simulink model "talos_navigation"  (R2023a)
settings: Solver=FixedStepDiscrete  StartTime=0.0  StopTime=10.0  FixedStep=1/1000.0  RelTol=1e-3  EnableMultiTasking=on
undefined symbols (not defined in the file): accel, child_frame_id, child_frame_id_SL_Info, data, data_SL_Info, header, layout, transform, transforms, transforms_SL_Info
libraries: ros2lib x187, simulink x9, sharedTrackingLibrary x1
(part 2 of 3)

== system talos_navigation/Parameters/estimator ==
  estimator_bus : BusCreator  Inputs=17  OutDataTypeStr=Bus: talos_nav_params_estimator  NonVirtualBus=on
  gravitational_acceleration : ros2lib/Get Parameter  ParameterName=navigation__estimator__gravitational_acceleration  ParameterType=double  ParameterMaxArrayLength=16  ParameterInitialValue=9.8  SampleTime=1/10.0  ModelName=ros2lib  BlockId=ParamGet_ros2lib_196
  imu_acceleration_bias : Subsystem
  imu_acceleration_bias_density : ros2lib/Get Parameter  ParameterName=navigation__estimator__imu_acceleration_bias_density  ParameterType=double  ParameterMaxArrayLength=16  ParameterInitialValue=1e-07  SampleTime=1/10.0  ModelName=ros2lib  BlockId=ParamGet_ros2lib_196
  imu_acceleration_bias_rotation_variance : ros2lib/Get Parameter  ParameterName=navigation__estimator__imu_acceleration_bias_rotation_variance  ParameterType=double  ParameterMaxArrayLength=16  ParameterInitialValue=0.0016  SampleTime=1/10.0  ModelName=ros2lib  BlockId=ParamGet_ros2lib_196
  imu_acceleration_bias_variance : ros2lib/Get Parameter  ParameterName=navigation__estimator__imu_acceleration_bias_variance  ParameterType=double  ParameterMaxArrayLength=16  ParameterInitialValue=0.0004  SampleTime=1/10.0  ModelName=ros2lib  BlockId=ParamGet_ros2lib_196
  imu_acceleration_update : ros2lib/Get Parameter  ParameterName=navigation__estimator__imu_acceleration_update  ParameterType=int64  ParameterMaxArrayLength=16  ParameterInitialValue=2  SampleTime=1/10.0  ModelName=talos_navigation  BlockId=ParamGet_talos_navigation_167
  imu_angular_acceleration_noise_bandwidth : ros2lib/Get Parameter  ParameterName=navigation__estimator__imu_angular_acceleration_noise_bandwidth  ParameterType=double  ParameterMaxArrayLength=16  ParameterInitialValue=40  SampleTime=1/10.0  ModelName=ros2lib  BlockId=ParamGet_ros2lib_196
  imu_angular_acceleration_time_constant : ros2lib/Get Parameter  ParameterName=navigation__estimator__imu_angular_acceleration_time_constant  ParameterType=double  ParameterMaxArrayLength=16  ParameterInitialValue=0.005  SampleTime=1/10.0  ModelName=ros2lib  BlockId=ParamGet_ros2lib_196
  imu_quaternion_norm_tolerance : ros2lib/Get Parameter  ParameterName=navigation__estimator__imu_quaternion_norm_tolerance  ParameterType=double  ParameterMaxArrayLength=16  ParameterInitialValue=0.01  SampleTime=1/10.0  ModelName=ros2lib  BlockId=ParamGet_ros2lib_196
  imu_yaw_rate_fallback : ros2lib/Get Parameter  ParameterName=navigation__estimator__imu_yaw_rate_fallback  ParameterType=boolean  ParameterMaxArrayLength=16  ParameterInitialValue=1  SampleTime=1/10.0  ModelName=talos_navigation  BlockId=ParamGet_talos_navigation_219
  imu_yaw_rate_fallback_variance : ros2lib/Get Parameter  ParameterName=navigation__estimator__imu_yaw_rate_fallback_variance  ParameterType=double  ParameterMaxArrayLength=16  ParameterInitialValue=0.0001  SampleTime=1/10.0  ModelName=ros2lib  BlockId=ParamGet_ros2lib_196
  initial_quaternion_tolerance : ros2lib/Get Parameter  ParameterName=navigation__estimator__initial_quaternion_tolerance  ParameterType=double  ParameterMaxArrayLength=16  ParameterInitialValue=0.001  SampleTime=1/10.0  ModelName=ros2lib  BlockId=ParamGet_ros2lib_196
  initialize_tilt_from_imu : ros2lib/Get Parameter  ParameterName=navigation__estimator__initialize_tilt_from_imu  ParameterType=boolean  ParameterMaxArrayLength=16  ParameterInitialValue=1  SampleTime=1/10.0  ModelName=talos_navigation  BlockId=ParamGet_talos_navigation_165
  process_noise_diag : Subsystem
  reset_covariance_diag : Subsystem
  scalar_fog_correction : ros2lib/Get Parameter  ParameterName=navigation__estimator__scalar_fog_correction  ParameterType=boolean  ParameterMaxArrayLength=16  ParameterInitialValue=1  SampleTime=1/10.0  ModelName=talos_navigation  BlockId=ParamGet_talos_navigation_222
  vectornav_tilt_correction_frequency : ros2lib/Get Parameter  ParameterName=navigation__estimator__vectornav_tilt_correction_frequency  ParameterType=double  ParameterMaxArrayLength=16  ParameterInitialValue=0  SampleTime=1/10.0  ModelName=ros2lib  BlockId=ParamGet_ros2lib_196
  estimator : Outport
  wires:
  initialize_tilt_from_imu/1 -> estimator_bus/1  "initialize_tilt_from_imu"
  vectornav_tilt_correction_frequency/1 -> estimator_bus/2  "vectornav_tilt_correction_frequency"
  imu_acceleration_update/1 -> estimator_bus/3  "imu_acceleration_update"
  gravitational_acceleration/1 -> estimator_bus/4  "gravitational_acceleration"
  imu_acceleration_bias/1(value) -> estimator_bus/5  "imu_acceleration_bias"
  imu_acceleration_bias_density/1 -> estimator_bus/6  "imu_acceleration_bias_density"
  imu_acceleration_bias_variance/1 -> estimator_bus/7  "imu_acceleration_bias_variance"
  imu_acceleration_bias_rotation_variance/1 -> estimator_bus/8  "imu_acceleration_bias_rotation_variance"
  imu_angular_acceleration_time_constant/1 -> estimator_bus/9  "imu_angular_acceleration_time_constant"
  imu_angular_acceleration_noise_bandwidth/1 -> estimator_bus/10  "imu_angular_acceleration_noise_bandwidth"
  process_noise_diag/1(value) -> estimator_bus/11  "process_noise_diag"
  reset_covariance_diag/1(value) -> estimator_bus/12  "reset_covariance_diag"
  initial_quaternion_tolerance/1 -> estimator_bus/13  "initial_quaternion_tolerance"
  imu_yaw_rate_fallback/1 -> estimator_bus/14  "imu_yaw_rate_fallback"
  imu_yaw_rate_fallback_variance/1 -> estimator_bus/15  "imu_yaw_rate_fallback_variance"
  imu_quaternion_norm_tolerance/1 -> estimator_bus/16  "imu_quaternion_norm_tolerance"
  scalar_fog_correction/1 -> estimator_bus/17  "scalar_fog_correction"
  estimator_bus/1 -> estimator/1

== system talos_navigation/Parameters/frames ==
  base_link_frame : ros2lib/Get Parameter  ParameterName=navigation__frames__base_link_frame  ParameterType=uint8[]  ParameterMaxArrayLength=64  ParameterInitialValue=0.0  SampleTime=1/10.0  ModelName=talos_navigation  BlockId=ParamGet_talos_navigation_7
  base_link_frame_length : Terminator
  dvl_frame_fallback : ros2lib/Get Parameter  ParameterName=navigation__frames__dvl_frame_fallback  ParameterType=uint8[]  ParameterMaxArrayLength=64  ParameterInitialValue=0.0  SampleTime=1/10.0  ModelName=talos_navigation  BlockId=ParamGet_talos_navigation_14
  dvl_frame_fallback_length : Terminator
  fog_frame_fallback : ros2lib/Get Parameter  ParameterName=navigation__frames__fog_frame_fallback  ParameterType=uint8[]  ParameterMaxArrayLength=64  ParameterInitialValue=0.0  SampleTime=1/10.0  ModelName=talos_navigation  BlockId=ParamGet_talos_navigation_12
  fog_frame_fallback_length : Terminator
  frames_bus : BusCreator  Inputs=6  OutDataTypeStr=Bus: talos_nav_params_frames  NonVirtualBus=on
  imu_frame_fallback : ros2lib/Get Parameter  ParameterName=navigation__frames__imu_frame_fallback  ParameterType=uint8[]  ParameterMaxArrayLength=64  ParameterInitialValue=0.0  SampleTime=1/10.0  ModelName=talos_navigation  BlockId=ParamGet_talos_navigation_10
  imu_frame_fallback_length : Terminator
  publish_tf : ros2lib/Get Parameter  ParameterName=navigation__frames__publish_tf  ParameterType=boolean  ParameterMaxArrayLength=16  ParameterInitialValue=1  SampleTime=1/10.0  ModelName=talos_navigation  BlockId=ParamGet_talos_navigation_9
  world_frame : ros2lib/Get Parameter  ParameterName=navigation__frames__world_frame  ParameterType=uint8[]  ParameterMaxArrayLength=64  ParameterInitialValue=0.0  SampleTime=1/10.0  ModelName=talos_navigation  BlockId=ParamGet_talos_navigation_5
  world_frame_length : Terminator
  frames : Outport
  wires:
  world_frame/2 -> world_frame_length/1
  world_frame/1 -> frames_bus/1  "world_frame"
  base_link_frame/2 -> base_link_frame_length/1
  base_link_frame/1 -> frames_bus/2  "base_link_frame"
  publish_tf/1 -> frames_bus/3  "publish_tf"
  imu_frame_fallback/2 -> imu_frame_fallback_length/1
  imu_frame_fallback/1 -> frames_bus/4  "imu_frame_fallback"
  fog_frame_fallback/2 -> fog_frame_fallback_length/1
  fog_frame_fallback/1 -> frames_bus/5  "fog_frame_fallback"
  dvl_frame_fallback/2 -> dvl_frame_fallback_length/1
  dvl_frame_fallback/1 -> frames_bus/6  "dvl_frame_fallback"
  frames_bus/1 -> frames/1

== system talos_navigation/Parameters/gates ==
  depth_rejection_threshold : ros2lib/Get Parameter  ParameterName=navigation__gates__depth_rejection_threshold  ParameterType=double  ParameterMaxArrayLength=16  ParameterInitialValue=5  SampleTime=1/10.0  ModelName=ros2lib  BlockId=ParamGet_ros2lib_196
  dvl_frozen_sample_limit : ros2lib/Get Parameter  ParameterName=navigation__gates__dvl_frozen_sample_limit  ParameterType=int64  ParameterMaxArrayLength=16  ParameterInitialValue=4  SampleTime=1/10.0  ModelName=talos_navigation  BlockId=ParamGet_talos_navigation_240
  dvl_rejection_threshold : ros2lib/Get Parameter  ParameterName=navigation__gates__dvl_rejection_threshold  ParameterType=double  ParameterMaxArrayLength=16  ParameterInitialValue=5  SampleTime=1/10.0  ModelName=ros2lib  BlockId=ParamGet_ros2lib_196
  dvl_sigma_jump_ratio : ros2lib/Get Parameter  ParameterName=navigation__gates__dvl_sigma_jump_ratio  ParameterType=double  ParameterMaxArrayLength=16  ParameterInitialValue=2  SampleTime=1/10.0  ModelName=ros2lib  BlockId=ParamGet_ros2lib_196
  dvl_sigma_min_history : ros2lib/Get Parameter  ParameterName=navigation__gates__dvl_sigma_min_history  ParameterType=int64  ParameterMaxArrayLength=16  ParameterInitialValue=8  SampleTime=1/10.0  ModelName=talos_navigation  BlockId=ParamGet_talos_navigation_242
  fog_rejection_threshold : ros2lib/Get Parameter  ParameterName=navigation__gates__fog_rejection_threshold  ParameterType=double  ParameterMaxArrayLength=16  ParameterInitialValue=0  SampleTime=1/10.0  ModelName=ros2lib  BlockId=ParamGet_ros2lib_196
  fog_vn_rate_tolerance : ros2lib/Get Parameter  ParameterName=navigation__gates__fog_vn_rate_tolerance  ParameterType=double  ParameterMaxArrayLength=16  ParameterInitialValue=0.05  SampleTime=1/10.0  ModelName=ros2lib  BlockId=ParamGet_ros2lib_196
  gate_consistency_stddev : Subsystem
  gate_consistency_threshold : ros2lib/Get Parameter  ParameterName=navigation__gates__gate_consistency_threshold  ParameterType=double  ParameterMaxArrayLength=16  ParameterInitialValue=2.5  SampleTime=1/10.0  ModelName=ros2lib  BlockId=ParamGet_ros2lib_196
  gate_flap_factor : ros2lib/Get Parameter  ParameterName=navigation__gates__gate_flap_factor  ParameterType=double  ParameterMaxArrayLength=16  ParameterInitialValue=4  SampleTime=1/10.0  ModelName=ros2lib  BlockId=ParamGet_ros2lib_196
  gate_min_recovery_window : ros2lib/Get Parameter  ParameterName=navigation__gates__gate_min_recovery_window  ParameterType=double  ParameterMaxArrayLength=16  ParameterInitialValue=0.25  SampleTime=1/10.0  ModelName=ros2lib  BlockId=ParamGet_ros2lib_196
  gate_reacquire_max_scale : ros2lib/Get Parameter  ParameterName=navigation__gates__gate_reacquire_max_scale  ParameterType=double  ParameterMaxArrayLength=16  ParameterInitialValue=4  SampleTime=1/10.0  ModelName=ros2lib  BlockId=ParamGet_ros2lib_196
  gate_reacquire_samples : ros2lib/Get Parameter  ParameterName=navigation__gates__gate_reacquire_samples  ParameterType=int64  ParameterMaxArrayLength=16  ParameterInitialValue=4  SampleTime=1/10.0  ModelName=talos_navigation  BlockId=ParamGet_talos_navigation_245
  gate_recovery_samples : ros2lib/Get Parameter  ParameterName=navigation__gates__gate_recovery_samples  ParameterType=int64  ParameterMaxArrayLength=16  ParameterInitialValue=5  SampleTime=1/10.0  ModelName=talos_navigation  BlockId=ParamGet_talos_navigation_246
  gate_recovery_time : ros2lib/Get Parameter  ParameterName=navigation__gates__gate_recovery_time  ParameterType=double  ParameterMaxArrayLength=16  ParameterInitialValue=0.5  SampleTime=1/10.0  ModelName=ros2lib  BlockId=ParamGet_ros2lib_196
  gates_bus : BusCreator  Inputs=17  OutDataTypeStr=Bus: talos_nav_params_gates  NonVirtualBus=on
  tilt_rejection_threshold : ros2lib/Get Parameter  ParameterName=navigation__gates__tilt_rejection_threshold  ParameterType=double  ParameterMaxArrayLength=16  ParameterInitialValue=10  SampleTime=1/10.0  ModelName=ros2lib  BlockId=ParamGet_ros2lib_196
  vn_rate_pairing_window : ros2lib/Get Parameter  ParameterName=navigation__gates__vn_rate_pairing_window  ParameterType=double  ParameterMaxArrayLength=16  ParameterInitialValue=0.01  SampleTime=1/10.0  ModelName=ros2lib  BlockId=ParamGet_ros2lib_196
  gates : Outport
  wires:
  dvl_rejection_threshold/1 -> gates_bus/1  "dvl_rejection_threshold"
  depth_rejection_threshold/1 -> gates_bus/2  "depth_rejection_threshold"
  tilt_rejection_threshold/1 -> gates_bus/3  "tilt_rejection_threshold"
  fog_rejection_threshold/1 -> gates_bus/4  "fog_rejection_threshold"
  fog_vn_rate_tolerance/1 -> gates_bus/5  "fog_vn_rate_tolerance"
  vn_rate_pairing_window/1 -> gates_bus/6  "vn_rate_pairing_window"
  gate_recovery_time/1 -> gates_bus/7  "gate_recovery_time"
  gate_consistency_stddev/1(value) -> gates_bus/8  "gate_consistency_stddev"
  dvl_frozen_sample_limit/1 -> gates_bus/9  "dvl_frozen_sample_limit"
  dvl_sigma_jump_ratio/1 -> gates_bus/10  "dvl_sigma_jump_ratio"
  dvl_sigma_min_history/1 -> gates_bus/11  "dvl_sigma_min_history"
  gate_reacquire_max_scale/1 -> gates_bus/12  "gate_reacquire_max_scale"
  gate_consistency_threshold/1 -> gates_bus/13  "gate_consistency_threshold"
  gate_reacquire_samples/1 -> gates_bus/14  "gate_reacquire_samples"
  gate_recovery_samples/1 -> gates_bus/15  "gate_recovery_samples"
  gate_min_recovery_window/1 -> gates_bus/16  "gate_min_recovery_window"
  gate_flap_factor/1 -> gates_bus/17  "gate_flap_factor"
  gates_bus/1 -> gates/1

== system talos_navigation/Parameters/mounts ==
  depth_frame : ros2lib/Get Parameter  ParameterName=navigation__mounts__depth_frame  ParameterType=uint8[]  ParameterMaxArrayLength=64  ParameterInitialValue=0.0  SampleTime=1/10.0  ModelName=talos_navigation  BlockId=ParamGet_talos_navigation_62
  depth_frame_length : Terminator
  depth_mount_valid : ros2lib/Get Parameter  ParameterName=navigation__mounts__depth_mount_valid  ParameterType=boolean  ParameterMaxArrayLength=16  ParameterInitialValue=0  SampleTime=1/10.0  ModelName=talos_navigation  BlockId=ParamGet_talos_navigation_64
  depth_rotation : Subsystem
  depth_translation : Subsystem
  dvl_mount_valid : ros2lib/Get Parameter  ParameterName=navigation__mounts__dvl_mount_valid  ParameterType=boolean  ParameterMaxArrayLength=16  ParameterInitialValue=0  SampleTime=1/10.0  ModelName=talos_navigation  BlockId=ParamGet_talos_navigation_48
  dvl_rotation : Subsystem
  dvl_translation : Subsystem
  fog_mount_valid : ros2lib/Get Parameter  ParameterName=navigation__mounts__fog_mount_valid  ParameterType=boolean  ParameterMaxArrayLength=16  ParameterInitialValue=0  SampleTime=1/10.0  ModelName=talos_navigation  BlockId=ParamGet_talos_navigation_34
  fog_rotation : Subsystem
  fog_translation : Subsystem
  imu_mount_valid : ros2lib/Get Parameter  ParameterName=navigation__mounts__imu_mount_valid  ParameterType=boolean  ParameterMaxArrayLength=16  ParameterInitialValue=0  SampleTime=1/10.0  ModelName=talos_navigation  BlockId=ParamGet_talos_navigation_20
  imu_rotation : Subsystem
  imu_translation : Subsystem
  mounts_bus : BusCreator  Inputs=14  OutDataTypeStr=Bus: talos_nav_params_mounts  NonVirtualBus=on
  parameters_loaded : ros2lib/Get Parameter  ParameterName=navigation__mounts__parameters_loaded  ParameterType=boolean  ParameterMaxArrayLength=16  ParameterInitialValue=0  SampleTime=1/10.0  ModelName=talos_navigation  BlockId=ParamGet_talos_navigation_19
  mounts : Outport
  wires:
  parameters_loaded/1 -> mounts_bus/1  "parameters_loaded"
  imu_mount_valid/1 -> mounts_bus/2  "imu_mount_valid"
  imu_translation/1(value) -> mounts_bus/3  "imu_translation"
  imu_rotation/1(value) -> mounts_bus/4  "imu_rotation"
  fog_mount_valid/1 -> mounts_bus/5  "fog_mount_valid"
  fog_translation/1(value) -> mounts_bus/6  "fog_translation"
  fog_rotation/1(value) -> mounts_bus/7  "fog_rotation"
  dvl_mount_valid/1 -> mounts_bus/8  "dvl_mount_valid"
  dvl_translation/1(value) -> mounts_bus/9  "dvl_translation"
  dvl_rotation/1(value) -> mounts_bus/10  "dvl_rotation"
  depth_frame/2 -> depth_frame_length/1
  depth_frame/1 -> mounts_bus/11  "depth_frame"
  depth_mount_valid/1 -> mounts_bus/12  "depth_mount_valid"
  depth_translation/1(value) -> mounts_bus/13  "depth_translation"
  depth_rotation/1(value) -> mounts_bus/14  "depth_rotation"
  mounts_bus/1 -> mounts/1

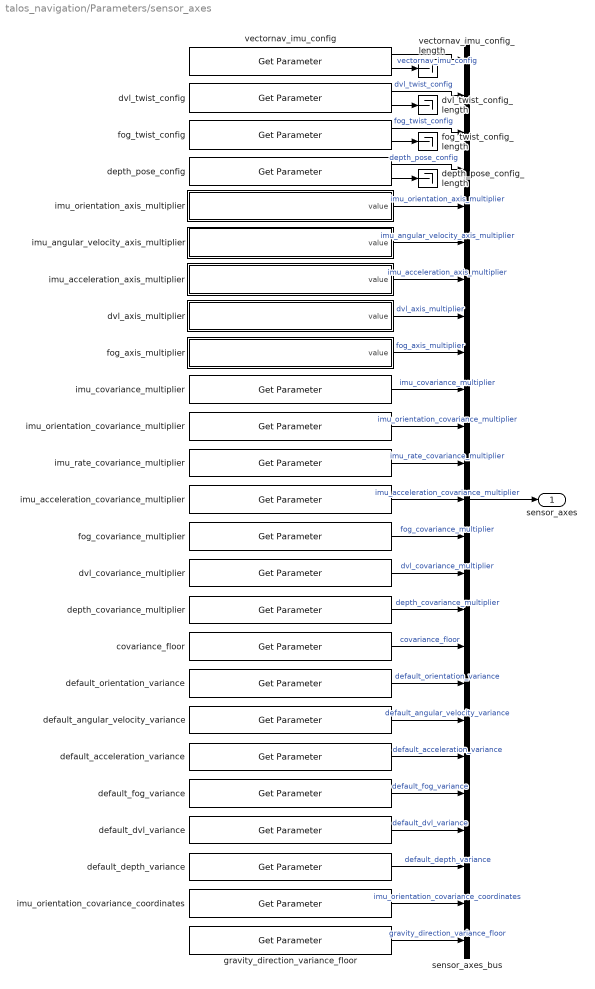
== system talos_navigation/Parameters/sensor_axes ==
  covariance_floor : ros2lib/Get Parameter  ParameterName=navigation__sensor_axes__covariance_floor  ParameterType=double  ParameterMaxArrayLength=16  ParameterInitialValue=1e-09  SampleTime=1/10.0  ModelName=ros2lib  BlockId=ParamGet_ros2lib_196
  default_acceleration_variance : ros2lib/Get Parameter  ParameterName=navigation__sensor_axes__default_acceleration_variance  ParameterType=double  ParameterMaxArrayLength=16  ParameterInitialValue=0.002  SampleTime=1/10.0  ModelName=ros2lib  BlockId=ParamGet_ros2lib_196
  default_angular_velocity_variance : ros2lib/Get Parameter  ParameterName=navigation__sensor_axes__default_angular_velocity_variance  ParameterType=double  ParameterMaxArrayLength=16  ParameterInitialValue=2e-05  SampleTime=1/10.0  ModelName=ros2lib  BlockId=ParamGet_ros2lib_196
  default_depth_variance : ros2lib/Get Parameter  ParameterName=navigation__sensor_axes__default_depth_variance  ParameterType=double  ParameterMaxArrayLength=16  ParameterInitialValue=0.0025  SampleTime=1/10.0  ModelName=ros2lib  BlockId=ParamGet_ros2lib_196
  default_dvl_variance : ros2lib/Get Parameter  ParameterName=navigation__sensor_axes__default_dvl_variance  ParameterType=double  ParameterMaxArrayLength=16  ParameterInitialValue=0.00025  SampleTime=1/10.0  ModelName=ros2lib  BlockId=ParamGet_ros2lib_196
  default_fog_variance : ros2lib/Get Parameter  ParameterName=navigation__sensor_axes__default_fog_variance  ParameterType=double  ParameterMaxArrayLength=16  ParameterInitialValue=1e-06  SampleTime=1/10.0  ModelName=ros2lib  BlockId=ParamGet_ros2lib_196
  default_orientation_variance : ros2lib/Get Parameter  ParameterName=navigation__sensor_axes__default_orientation_variance  ParameterType=double  ParameterMaxArrayLength=16  ParameterInitialValue=0.0002  SampleTime=1/10.0  ModelName=ros2lib  BlockId=ParamGet_ros2lib_196
  depth_covariance_multiplier : ros2lib/Get Parameter  ParameterName=navigation__sensor_axes__depth_covariance_multiplier  ParameterType=double  ParameterMaxArrayLength=16  ParameterInitialValue=1  SampleTime=1/10.0  ModelName=ros2lib  BlockId=ParamGet_ros2lib_196
  depth_pose_config : ros2lib/Get Parameter  ParameterName=navigation__sensor_axes__depth_pose_config  ParameterType=boolean[]  ParameterMaxArrayLength=15  ParameterInitialValue=[0;0;1;0;0;0;0;0;0;0;0;0;0;0;0]  SampleTime=1/10.0  ModelName=talos_navigation  BlockId=ParamGet_talos_navigation_114
  depth_pose_config_length : Terminator
  dvl_axis_multiplier : Subsystem
  dvl_covariance_multiplier : ros2lib/Get Parameter  ParameterName=navigation__sensor_axes__dvl_covariance_multiplier  ParameterType=double  ParameterMaxArrayLength=16  ParameterInitialValue=1  SampleTime=1/10.0  ModelName=ros2lib  BlockId=ParamGet_ros2lib_196
  dvl_twist_config : ros2lib/Get Parameter  ParameterName=navigation__sensor_axes__dvl_twist_config  ParameterType=boolean[]  ParameterMaxArrayLength=15  ParameterInitialValue=[0;0;0;0;0;0;1;1;1;0;0;0;0;0;0]  SampleTime=1/10.0  ModelName=talos_navigation  BlockId=ParamGet_talos_navigation_110
  dvl_twist_config_length : Terminator
  fog_axis_multiplier : Subsystem
  fog_covariance_multiplier : ros2lib/Get Parameter  ParameterName=navigation__sensor_axes__fog_covariance_multiplier  ParameterType=double  ParameterMaxArrayLength=16  ParameterInitialValue=1  SampleTime=1/10.0  ModelName=ros2lib  BlockId=ParamGet_ros2lib_196
  fog_twist_config : ros2lib/Get Parameter  ParameterName=navigation__sensor_axes__fog_twist_config  ParameterType=boolean[]  ParameterMaxArrayLength=15  ParameterInitialValue=[0;0;0;0;0;0;0;0;0;0;0;1;0;0;0]  SampleTime=1/10.0  ModelName=talos_navigation  BlockId=ParamGet_talos_navigation_112
  fog_twist_config_length : Terminator
  gravity_direction_variance_floor : ros2lib/Get Parameter  ParameterName=navigation__sensor_axes__gravity_direction_variance_floor  ParameterType=double  ParameterMaxArrayLength=16  ParameterInitialValue=1e-09  SampleTime=1/10.0  ModelName=ros2lib  BlockId=ParamGet_ros2lib_196
  imu_acceleration_axis_multiplier : Subsystem
  imu_acceleration_covariance_multiplier : ros2lib/Get Parameter  ParameterName=navigation__sensor_axes__imu_acceleration_covariance_multiplier  ParameterType=double  ParameterMaxArrayLength=16  ParameterInitialValue=1  SampleTime=1/10.0  ModelName=ros2lib  BlockId=ParamGet_ros2lib_196
  imu_angular_velocity_axis_multiplier : Subsystem
  imu_covariance_multiplier : ros2lib/Get Parameter  ParameterName=navigation__sensor_axes__imu_covariance_multiplier  ParameterType=double  ParameterMaxArrayLength=16  ParameterInitialValue=1  SampleTime=1/10.0  ModelName=ros2lib  BlockId=ParamGet_ros2lib_196
  imu_orientation_axis_multiplier : Subsystem
  imu_orientation_covariance_coordinates : ros2lib/Get Parameter  ParameterName=navigation__sensor_axes__imu_orientation_covariance_coordinates  ParameterType=int64  ParameterMaxArrayLength=16  ParameterInitialValue=1  SampleTime=1/10.0  ModelName=talos_navigation  BlockId=ParamGet_talos_navigation_160
  imu_orientation_covariance_multiplier : ros2lib/Get Parameter  ParameterName=navigation__sensor_axes__imu_orientation_covariance_multiplier  ParameterType=double  ParameterMaxArrayLength=16  ParameterInitialValue=1  SampleTime=1/10.0  ModelName=ros2lib  BlockId=ParamGet_ros2lib_196
  imu_rate_covariance_multiplier : ros2lib/Get Parameter  ParameterName=navigation__sensor_axes__imu_rate_covariance_multiplier  ParameterType=double  ParameterMaxArrayLength=16  ParameterInitialValue=0.01  SampleTime=1/10.0  ModelName=ros2lib  BlockId=ParamGet_ros2lib_196
  sensor_axes_bus : BusCreator  Inputs=25  OutDataTypeStr=Bus: talos_nav_params_sensor_axes  NonVirtualBus=on
  vectornav_imu_config : ros2lib/Get Parameter  ParameterName=navigation__sensor_axes__vectornav_imu_config  ParameterType=boolean[]  ParameterMaxArrayLength=15  ParameterInitialValue=[0;0;0;1;1;0;0;0;0;1;1;0;1;1;1]  SampleTime=1/10.0  ModelName=talos_navigation  BlockId=ParamGet_talos_navigation_108
  vectornav_imu_config_length : Terminator
  sensor_axes : Outport
  wires:
  vectornav_imu_config/2 -> vectornav_imu_config_length/1
  vectornav_imu_config/1 -> sensor_axes_bus/1  "vectornav_imu_config"
  dvl_twist_config/2 -> dvl_twist_config_length/1
  dvl_twist_config/1 -> sensor_axes_bus/2  "dvl_twist_config"
  fog_twist_config/2 -> fog_twist_config_length/1
  fog_twist_config/1 -> sensor_axes_bus/3  "fog_twist_config"
  depth_pose_config/2 -> depth_pose_config_length/1
  depth_pose_config/1 -> sensor_axes_bus/4  "depth_pose_config"
  imu_orientation_axis_multiplier/1(value) -> sensor_axes_bus/5  "imu_orientation_axis_multiplier"
  imu_angular_velocity_axis_multiplier/1(value) -> sensor_axes_bus/6  "imu_angular_velocity_axis_multiplier"
  imu_acceleration_axis_multiplier/1(value) -> sensor_axes_bus/7  "imu_acceleration_axis_multiplier"
  dvl_axis_multiplier/1(value) -> sensor_axes_bus/8  "dvl_axis_multiplier"
  fog_axis_multiplier/1(value) -> sensor_axes_bus/9  "fog_axis_multiplier"
  imu_covariance_multiplier/1 -> sensor_axes_bus/10  "imu_covariance_multiplier"
  imu_orientation_covariance_multiplier/1 -> sensor_axes_bus/11  "imu_orientation_covariance_multiplier"
  imu_rate_covariance_multiplier/1 -> sensor_axes_bus/12  "imu_rate_covariance_multiplier"
  imu_acceleration_covariance_multiplier/1 -> sensor_axes_bus/13  "imu_acceleration_covariance_multiplier"
  fog_covariance_multiplier/1 -> sensor_axes_bus/14  "fog_covariance_multiplier"
  dvl_covariance_multiplier/1 -> sensor_axes_bus/15  "dvl_covariance_multiplier"
  depth_covariance_multiplier/1 -> sensor_axes_bus/16  "depth_covariance_multiplier"
  covariance_floor/1 -> sensor_axes_bus/17  "covariance_floor"
  default_orientation_variance/1 -> sensor_axes_bus/18  "default_orientation_variance"
  default_angular_velocity_variance/1 -> sensor_axes_bus/19  "default_angular_velocity_variance"
  default_acceleration_variance/1 -> sensor_axes_bus/20  "default_acceleration_variance"
  default_fog_variance/1 -> sensor_axes_bus/21  "default_fog_variance"
  default_dvl_variance/1 -> sensor_axes_bus/22  "default_dvl_variance"
  default_depth_variance/1 -> sensor_axes_bus/23  "default_depth_variance"
  imu_orientation_covariance_coordinates/1 -> sensor_axes_bus/24  "imu_orientation_covariance_coordinates"
  gravity_direction_variance_floor/1 -> sensor_axes_bus/25  "gravity_direction_variance_floor"
  sensor_axes_bus/1 -> sensor_axes/1

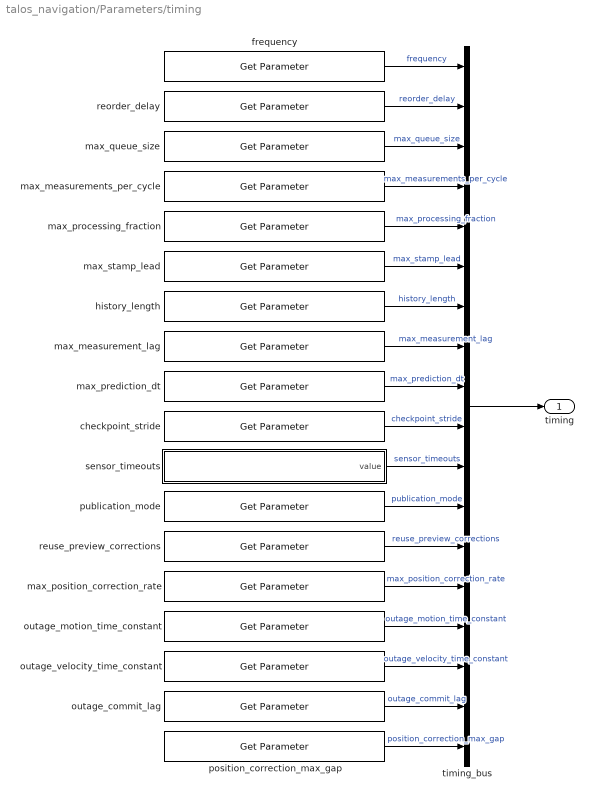
== system talos_navigation/Parameters/timing ==
  checkpoint_stride : ros2lib/Get Parameter  ParameterName=navigation__timing__checkpoint_stride  ParameterType=double  ParameterMaxArrayLength=16  ParameterInitialValue=0.005  SampleTime=1/10.0  ModelName=ros2lib  BlockId=ParamGet_ros2lib_196
  frequency : ros2lib/Get Parameter  ParameterName=navigation__timing__frequency  ParameterType=double  ParameterMaxArrayLength=16  ParameterInitialValue=30  SampleTime=1/10.0  ModelName=ros2lib  BlockId=ParamGet_ros2lib_196
  history_length : ros2lib/Get Parameter  ParameterName=navigation__timing__history_length  ParameterType=double  ParameterMaxArrayLength=16  ParameterInitialValue=0.5  SampleTime=1/10.0  ModelName=ros2lib  BlockId=ParamGet_ros2lib_196
  max_measurement_lag : ros2lib/Get Parameter  ParameterName=navigation__timing__max_measurement_lag  ParameterType=double  ParameterMaxArrayLength=16  ParameterInitialValue=2  SampleTime=1/10.0  ModelName=ros2lib  BlockId=ParamGet_ros2lib_196
  max_measurements_per_cycle : ros2lib/Get Parameter  ParameterName=navigation__timing__max_measurements_per_cycle  ParameterType=int64  ParameterMaxArrayLength=16  ParameterInitialValue=0  SampleTime=1/10.0  ModelName=talos_navigation  BlockId=ParamGet_talos_navigation_84
  max_position_correction_rate : ros2lib/Get Parameter  ParameterName=navigation__timing__max_position_correction_rate  ParameterType=double  ParameterMaxArrayLength=16  ParameterInitialValue=0.2  SampleTime=1/10.0  ModelName=ros2lib  BlockId=ParamGet_ros2lib_196
  max_prediction_dt : ros2lib/Get Parameter  ParameterName=navigation__timing__max_prediction_dt  ParameterType=double  ParameterMaxArrayLength=16  ParameterInitialValue=0.1  SampleTime=1/10.0  ModelName=ros2lib  BlockId=ParamGet_ros2lib_196
  max_processing_fraction : ros2lib/Get Parameter  ParameterName=navigation__timing__max_processing_fraction  ParameterType=double  ParameterMaxArrayLength=16  ParameterInitialValue=0.5  SampleTime=1/10.0  ModelName=ros2lib  BlockId=ParamGet_ros2lib_196
  max_queue_size : ros2lib/Get Parameter  ParameterName=navigation__timing__max_queue_size  ParameterType=int64  ParameterMaxArrayLength=16  ParameterInitialValue=512  SampleTime=1/10.0  ModelName=talos_navigation  BlockId=ParamGet_talos_navigation_83
  max_stamp_lead : ros2lib/Get Parameter  ParameterName=navigation__timing__max_stamp_lead  ParameterType=double  ParameterMaxArrayLength=16  ParameterInitialValue=1  SampleTime=1/10.0  ModelName=ros2lib  BlockId=ParamGet_ros2lib_196
  outage_commit_lag : ros2lib/Get Parameter  ParameterName=navigation__timing__outage_commit_lag  ParameterType=double  ParameterMaxArrayLength=16  ParameterInitialValue=1  SampleTime=1/10.0  ModelName=ros2lib  BlockId=ParamGet_ros2lib_196
  outage_motion_time_constant : ros2lib/Get Parameter  ParameterName=navigation__timing__outage_motion_time_constant  ParameterType=double  ParameterMaxArrayLength=16  ParameterInitialValue=0.5  SampleTime=1/10.0  ModelName=ros2lib  BlockId=ParamGet_ros2lib_196
  outage_velocity_time_constant : ros2lib/Get Parameter  ParameterName=navigation__timing__outage_velocity_time_constant  ParameterType=double  ParameterMaxArrayLength=16  ParameterInitialValue=2  SampleTime=1/10.0  ModelName=ros2lib  BlockId=ParamGet_ros2lib_196
  position_correction_max_gap : ros2lib/Get Parameter  ParameterName=navigation__timing__position_correction_max_gap  ParameterType=double  ParameterMaxArrayLength=16  ParameterInitialValue=1  SampleTime=1/10.0  ModelName=ros2lib  BlockId=ParamGet_ros2lib_196
  publication_mode : ros2lib/Get Parameter  ParameterName=navigation__timing__publication_mode  ParameterType=int64  ParameterMaxArrayLength=16  ParameterInitialValue=2  SampleTime=1/10.0  ModelName=talos_navigation  BlockId=ParamGet_talos_navigation_98
  reorder_delay : ros2lib/Get Parameter  ParameterName=navigation__timing__reorder_delay  ParameterType=double  ParameterMaxArrayLength=16  ParameterInitialValue=0.02  SampleTime=1/10.0  ModelName=ros2lib  BlockId=ParamGet_ros2lib_196
  reuse_preview_corrections : ros2lib/Get Parameter  ParameterName=navigation__timing__reuse_preview_corrections  ParameterType=boolean  ParameterMaxArrayLength=16  ParameterInitialValue=1  SampleTime=1/10.0  ModelName=talos_navigation  BlockId=ParamGet_talos_navigation_99
  sensor_timeouts : Subsystem
  timing_bus : BusCreator  Inputs=18  OutDataTypeStr=Bus: talos_nav_params_timing  NonVirtualBus=on
  timing : Outport
  wires:
  frequency/1 -> timing_bus/1  "frequency"
  reorder_delay/1 -> timing_bus/2  "reorder_delay"
  max_queue_size/1 -> timing_bus/3  "max_queue_size"
  max_measurements_per_cycle/1 -> timing_bus/4  "max_measurements_per_cycle"
  max_processing_fraction/1 -> timing_bus/5  "max_processing_fraction"
  max_stamp_lead/1 -> timing_bus/6  "max_stamp_lead"
  history_length/1 -> timing_bus/7  "history_length"
  max_measurement_lag/1 -> timing_bus/8  "max_measurement_lag"
  max_prediction_dt/1 -> timing_bus/9  "max_prediction_dt"
  checkpoint_stride/1 -> timing_bus/10  "checkpoint_stride"
  sensor_timeouts/1(value) -> timing_bus/11  "sensor_timeouts"
  publication_mode/1 -> timing_bus/12  "publication_mode"
  reuse_preview_corrections/1 -> timing_bus/13  "reuse_preview_corrections"
  max_position_correction_rate/1 -> timing_bus/14  "max_position_correction_rate"
  outage_motion_time_constant/1 -> timing_bus/15  "outage_motion_time_constant"
  outage_velocity_time_constant/1 -> timing_bus/16  "outage_velocity_time_constant"
  outage_commit_lag/1 -> timing_bus/17  "outage_commit_lag"
  position_correction_max_gap/1 -> timing_bus/18  "position_correction_max_gap"
  timing_bus/1 -> timing/1

== system talos_navigation/Publish_System/Acceleration ==
  enable : Inport
  time : Inport  Port=2
  base_id : Inport  Port=3
  base_length : Inport  Port=4
  x : Inport  Port=5
  accel_cov : Inport  Port=6
  blank : ros2lib/Blank Message  messageClass=Message  entityType=geometry_msgs/AccelWithCovarianceStamped  messageType=geometry_msgs/AccelWithCovarianceStamped  SampleTime=1/500.0
  fill : BusAssignment  AssignedSignals=header.stamp,header.frame_id,header.frame_id_SL_Info.CurrentLength,accel.accel.linear.x,accel.accel.linear.y,accel.accel.linear.z,accel.covariance
  fill_publish : Subsystem  TreatAsAtomicUnit=on
  x_elements : Demux  Outputs=3
  x_fields : Selector  InputPortWidth=19  IndexOptions=Index vector (dialog)  Indices=14:16  OutputSizes=1
  wires:
  blank/1 -> fill/1
  time/1 -> fill/2  "header.stamp"
  base_id/1 -> fill/3  "header.frame_id"
  base_length/1 -> fill/4  "frame_id_SL_Info.CurrentLength"
  x/1 -> x_fields/1
  x_fields/1 -> x_elements/1
  x_elements/1 -> fill/5  "linear.x"
  x_elements/2 -> fill/6  "linear.y"
  x_elements/3 -> fill/7  "linear.z"
  accel_cov/1 -> fill/8  "accel.covariance"
  fill/1 -> fill_publish/1(msg)  "msg"
  enable/1 -> fill_publish/Enable

== system talos_navigation/Publish_System/Base_Frame_ID ==
  name : Inport
  chars : Sum  Inputs=+  OutDataTypeStr=uint32
  count : DataTypeConversion  OutDataTypeStr=uint32  SaturateOnIntegerOverflow=off  RndMeth=Floor
  is_char : simulink/Logic and Bit Operations/Compare To Zero  relop=~=  OutDataTypeStr=boolean
  padded : Concatenate
  padding : Constant  Value=zeros(64, 1, 'uint8')
  frame_id : Outport
  length : Outport  Port=2
  wires:
  name/1 -> padded/1, is_char/1
  padding/1 -> padded/2
  padded/1 -> frame_id/1  "frame_id"
  is_char/1 -> count/1
  count/1 -> chars/1
  chars/1 -> length/1  "length"

== system talos_navigation/Publish_System/Diagnostics ==
  enable : Inport
  diag : Inport  Port=2
  part_0_blank : ros2lib/Blank Message  messageClass=Message  entityType=std_msgs/Float64MultiArray  messageType=std_msgs/Float64MultiArray  SampleTime=1/500.0
  part_0_fill : BusAssignment  AssignedSignals=data,data_SL_Info.CurrentLength,layout.data_offset
  part_0_length : Constant  Value=uint32(128)  OutDataTypeStr=uint32
  part_0_offset : Constant  Value=uint32(0)  OutDataTypeStr=uint32
  part_0_publish : Subsystem  TreatAsAtomicUnit=on
  part_0_values : Selector  InputPortWidth=162  IndexOptions=Starting index (dialog)  Indices=1  OutputSizes=128
  part_1_blank : ros2lib/Blank Message  messageClass=Message  entityType=std_msgs/Float64MultiArray  messageType=std_msgs/Float64MultiArray  SampleTime=1/500.0
  part_1_data : Concatenate
  part_1_fill : BusAssignment  AssignedSignals=data,data_SL_Info.CurrentLength,layout.data_offset
  part_1_length : Constant  Value=uint32(62)  OutDataTypeStr=uint32
  part_1_offset : Constant  Value=uint32(100)  OutDataTypeStr=uint32
  part_1_padding : Constant  Value=zeros(66, 1)
  part_1_publish : Subsystem  TreatAsAtomicUnit=on
  part_1_values : Selector  InputPortWidth=162  IndexOptions=Starting index (dialog)  Indices=101  OutputSizes=62
  wires:
  part_0_blank/1 -> part_0_fill/1
  part_0_length/1 -> part_0_fill/3  "length"
  part_0_offset/1 -> part_0_fill/4  "offset"
  [Diag] -> part_0_values/1
  part_0_values/1 -> part_0_fill/2  "data"
  part_0_fill/1 -> part_0_publish/1(msg)  "msg"
  enable/1 -> part_0_publish/Enable, part_1_publish/Enable
  part_1_blank/1 -> part_1_fill/1
  part_1_length/1 -> part_1_fill/3  "length"
  part_1_offset/1 -> part_1_fill/4  "offset"
  [Diag] -> part_1_values/1
  part_1_values/1 -> part_1_data/1
  part_1_padding/1 -> part_1_data/2
  part_1_data/1 -> part_1_fill/2  "data"
  part_1_fill/1 -> part_1_publish/1(msg)  "msg"
  diag/1 -> [Diag]

== system talos_navigation/Publish_System/Odometry ==
  enable : Inport
  time : Inport  Port=2
  world_id : Inport  Port=3
  world_length : Inport  Port=4
  base_id : Inport  Port=5
  base_length : Inport  Port=6
  x : Inport  Port=7
  pose_cov : Inport  Port=8
  twist_cov : Inport  Port=9
  blank : ros2lib/Blank Message  messageClass=Message  entityType=nav_msgs/Odometry  messageType=nav_msgs/Odometry  SampleTime=1/500.0
  fill : BusAssignment  AssignedSignals=header.stamp,header.frame_id,header.frame_id_SL_Info.CurrentLength,child_frame_id,child_frame_id_SL_Info.CurrentLength,pose.pose.position.x,pose.pose.position.y,pose.pose.position.z,pose.pose.orientation.w,pose.pose.orientation.x,pose.pose.orientation.y,pose.pose.orientation.z,twist.twist.linear.x,twist.twist.linear.y,twist.twist.linear.z,twist.twist.angular.x,twist.twist.angular.y,twist.twist.angular.z,pose.covariance,twist.covariance
  fill_publish : Subsystem  TreatAsAtomicUnit=on
  x_elements : Demux  Outputs=13
  x_fields : Selector  InputPortWidth=19  IndexOptions=Index vector (dialog)  Indices=1:13  OutputSizes=1
  wires:
  blank/1 -> fill/1
  time/1 -> fill/2  "header.stamp"
  world_id/1 -> fill/3  "header.frame_id"
  world_length/1 -> fill/4  "frame_id_SL_Info.CurrentLength"
  base_id/1 -> fill/5  "child_frame_id"
  base_length/1 -> fill/6  "child_frame_id_SL_Info.CurrentLength"
  x/1 -> x_fields/1
  x_fields/1 -> x_elements/1
  x_elements/1 -> fill/7  "position.x"
  x_elements/2 -> fill/8  "position.y"
  x_elements/3 -> fill/9  "position.z"
  x_elements/4 -> fill/10  "orientation.w"
  x_elements/5 -> fill/11  "orientation.x"
  x_elements/6 -> fill/12  "orientation.y"
  x_elements/7 -> fill/13  "orientation.z"
  x_elements/8 -> fill/14  "linear.x"
  x_elements/9 -> fill/15  "linear.y"
  x_elements/10 -> fill/16  "linear.z"
  x_elements/11 -> fill/17  "angular.x"
  x_elements/12 -> fill/18  "angular.y"
  x_elements/13 -> fill/19  "angular.z"
  pose_cov/1 -> fill/20  "pose.covariance"
  twist_cov/1 -> fill/21  "twist.covariance"
  fill/1 -> fill_publish/1(msg)  "msg"
  enable/1 -> fill_publish/Enable

== system talos_navigation/Publish_System/TF ==
  enable : Inport
  time : Inport  Port=2
  world_id : Inport  Port=3
  world_length : Inport  Port=4
  base_id : Inport  Port=5
  base_length : Inport  Port=6
  x : Inport  Port=7
  blank : ros2lib/Blank Message  messageClass=Message  entityType=geometry_msgs/TransformStamped  messageType=geometry_msgs/TransformStamped  SampleTime=1/500.0
  fill : BusAssignment  AssignedSignals=header.stamp,header.frame_id,header.frame_id_SL_Info.CurrentLength,child_frame_id,child_frame_id_SL_Info.CurrentLength,transform.translation.x,transform.translation.y,transform.translation.z,transform.rotation.w,transform.rotation.x,transform.rotation.y,transform.rotation.z
  first : Assignment  DiagnosticForDimensions=Warning  IndexOptions=Index vector (dialog)  Indices=1  OutputSizes=1
  one : Constant  Value=uint32(1)  OutDataTypeStr=uint32
  tf_blank : ros2lib/Blank Message  messageClass=Message  entityType=tf2_msgs/TFMessage  messageType=tf2_msgs/TFMessage  SampleTime=1/500.0
  tf_message : BusAssignment  AssignedSignals=transforms,transforms_SL_Info.CurrentLength
  tf_message_publish : Subsystem  TreatAsAtomicUnit=on
  transforms : BusSelector  OutputSignals=transforms
  x_elements : Demux  Outputs=7
  x_fields : Selector  InputPortWidth=19  IndexOptions=Index vector (dialog)  Indices=1:7  OutputSizes=1
  wires:
  blank/1 -> fill/1
  time/1 -> fill/2  "header.stamp"
  world_id/1 -> fill/3  "header.frame_id"
  world_length/1 -> fill/4  "frame_id_SL_Info.CurrentLength"
  base_id/1 -> fill/5  "child_frame_id"
  base_length/1 -> fill/6  "child_frame_id_SL_Info.CurrentLength"
  x/1 -> x_fields/1
  x_fields/1 -> x_elements/1
  x_elements/1 -> fill/7  "translation.x"
  x_elements/2 -> fill/8  "translation.y"
  x_elements/3 -> fill/9  "translation.z"
  x_elements/4 -> fill/10  "rotation.w"
  x_elements/5 -> fill/11  "rotation.x"
  x_elements/6 -> fill/12  "rotation.y"
  x_elements/7 -> fill/13  "rotation.z"
  tf_blank/1 -> tf_message/1, transforms/1
  transforms/1 -> first/1  "<transforms>"
  fill/1 -> first/2  "transform"
  first/1 -> tf_message/2  "transforms"
  one/1 -> tf_message/3  "count"
  tf_message/1 -> tf_message_publish/1(msg)  "msg"
  enable/1 -> tf_message_publish/Enable

== system talos_navigation/Publish_System/World_Frame_ID ==
  name : Inport
  chars : Sum  Inputs=+  OutDataTypeStr=uint32
  count : DataTypeConversion  OutDataTypeStr=uint32  SaturateOnIntegerOverflow=off  RndMeth=Floor
  is_char : simulink/Logic and Bit Operations/Compare To Zero  relop=~=  OutDataTypeStr=boolean
  padded : Concatenate
  padding : Constant  Value=zeros(64, 1, 'uint8')
  frame_id : Outport
  length : Outport  Port=2
  wires:
  name/1 -> padded/1, is_char/1
  padding/1 -> padded/2
  padded/1 -> frame_id/1  "frame_id"
  is_char/1 -> count/1
  count/1 -> chars/1
  chars/1 -> length/1  "length"

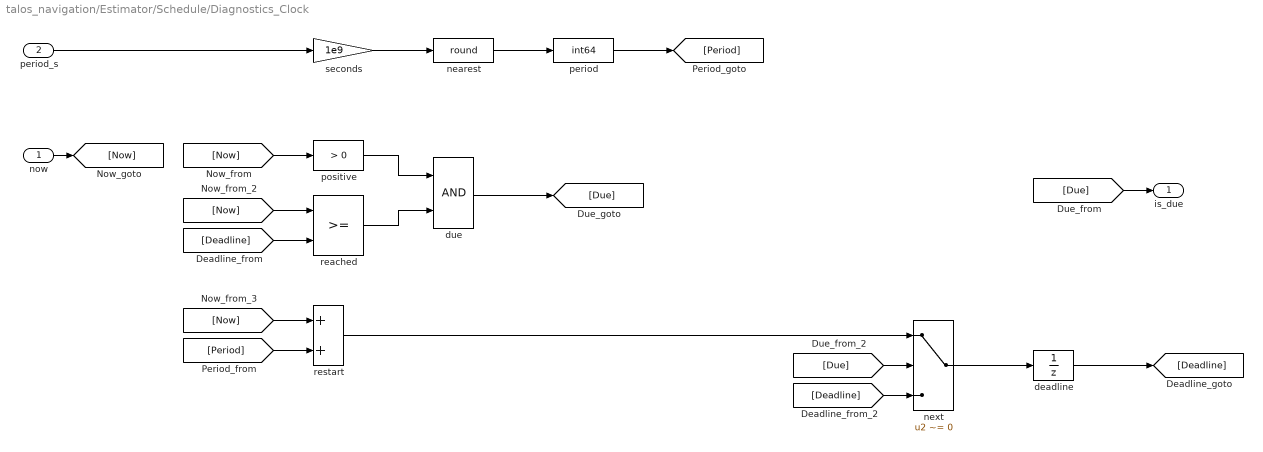
== system talos_navigation/Estimator/Schedule/Diagnostics_Clock ==
  now : Inport
  period_s : Inport  Port=2
  deadline : UnitDelay  InitialCondition=int64(0)  SampleTime=-1  HasFrameUpgradeWarning=on
  due : Logic  AllPortsSameDT=off  OutDataTypeStr=boolean
  nearest : Rounding  Operator=round
  next : Switch  Criteria=u2 ~= 0  SaturateOnIntegerOverflow=off  InputSameDT=off
  period : DataTypeConversion  OutDataTypeStr=int64  SaturateOnIntegerOverflow=off  RndMeth=Floor
  positive : simulink/Logic and Bit Operations/Compare To Zero  relop=>  OutDataTypeStr=boolean
  reached : RelationalOperator  OutDataTypeStr=boolean  RndMeth=Simplest  InputSameDT=off
  restart : Sum
  seconds : Gain  Gain=1e9
  is_due : Outport
  wires:
  period_s/1 -> seconds/1
  seconds/1 -> nearest/1
  nearest/1 -> period/1
  period/1 -> [Period]
  now/1 -> [Now]
  [Now] -> positive/1
  [Now] -> reached/1
  [Deadline] -> reached/2
  positive/1 -> due/1
  reached/1 -> due/2
  due/1 -> [Due]
  [Due] -> is_due/1
  [Now] -> restart/1
  [Period] -> restart/2
  restart/1 -> next/1
  [Due] -> next/2
  [Deadline] -> next/3
  next/1 -> deadline/1
  deadline/1 -> [Deadline]

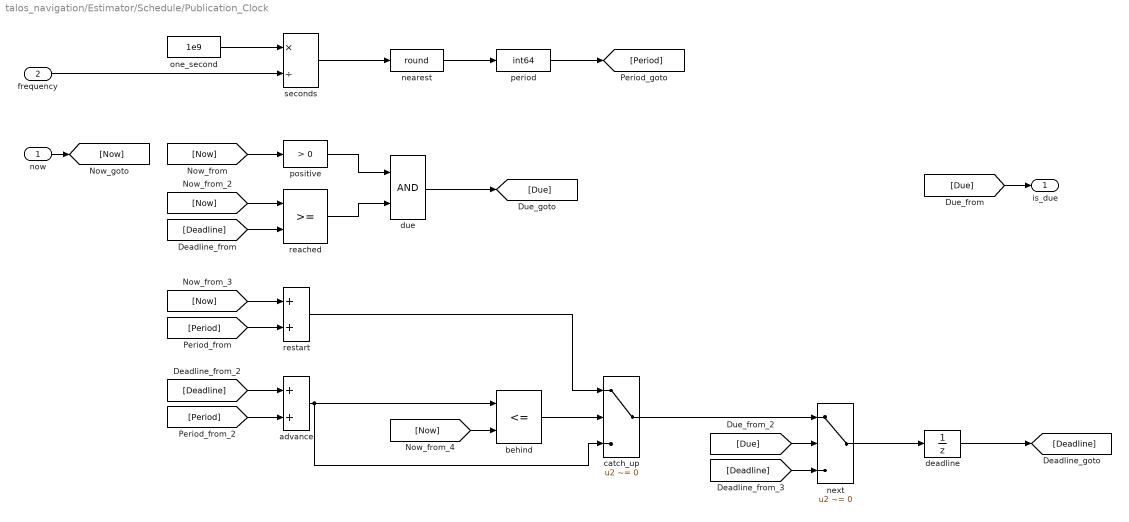
== system talos_navigation/Estimator/Schedule/Publication_Clock ==
  now : Inport
  frequency : Inport  Port=2
  advance : Sum
  behind : RelationalOperator  Operator=<=  OutDataTypeStr=boolean  RndMeth=Simplest  InputSameDT=off
  catch_up : Switch  Criteria=u2 ~= 0  SaturateOnIntegerOverflow=off  InputSameDT=off
  deadline : UnitDelay  InitialCondition=int64(0)  SampleTime=-1  HasFrameUpgradeWarning=on
  due : Logic  AllPortsSameDT=off  OutDataTypeStr=boolean
  nearest : Rounding  Operator=round
  next : Switch  Criteria=u2 ~= 0  SaturateOnIntegerOverflow=off  InputSameDT=off
  one_second : Constant  Value=1e9
  period : DataTypeConversion  OutDataTypeStr=int64  SaturateOnIntegerOverflow=off  RndMeth=Floor
  positive : simulink/Logic and Bit Operations/Compare To Zero  relop=>  OutDataTypeStr=boolean
  reached : RelationalOperator  OutDataTypeStr=boolean  RndMeth=Simplest  InputSameDT=off
  restart : Sum
  seconds : Product  Inputs=*/
  is_due : Outport
  wires:
  one_second/1 -> seconds/1
  frequency/1 -> seconds/2
  seconds/1 -> nearest/1
  nearest/1 -> period/1
  period/1 -> [Period]
  now/1 -> [Now]
  [Now] -> positive/1
  [Now] -> reached/1
  [Deadline] -> reached/2
  positive/1 -> due/1
  reached/1 -> due/2
  due/1 -> [Due]
  [Due] -> is_due/1
  [Now] -> restart/1
  [Period] -> restart/2
  [Deadline] -> advance/1
  [Period] -> advance/2
  [Now] -> behind/2
  advance/1 -> behind/1, catch_up/3
  restart/1 -> catch_up/1
  behind/1 -> catch_up/2
  catch_up/1 -> next/1
  [Due] -> next/2
  [Deadline] -> next/3
  next/1 -> deadline/1
  deadline/1 -> [Deadline]

== system talos_navigation/Measurement_Intake/DVL/stamp ==
  stamp : Inport
  nanosec_int64 : DataTypeConversion  OutDataTypeStr=int64  SaturateOnIntegerOverflow=off  RndMeth=Floor
  parts : BusSelector  OutputSignals=sec,nanosec
  per_second : Gain  Gain=1000000000  ParamDataTypeStr=int64  OutDataTypeStr=int64
  sec_int64 : DataTypeConversion  OutDataTypeStr=int64  SaturateOnIntegerOverflow=off  RndMeth=Floor
  total : Sum  OutDataTypeStr=int64
  ns : Outport
  wires:
  stamp/1 -> parts/1
  parts/1 -> sec_int64/1  "<sec>"
  parts/2 -> nanosec_int64/1  "<nanosec>"
  sec_int64/1 -> per_second/1
  per_second/1 -> total/1
  nanosec_int64/1 -> total/2
  total/1 -> ns/1  "ns"

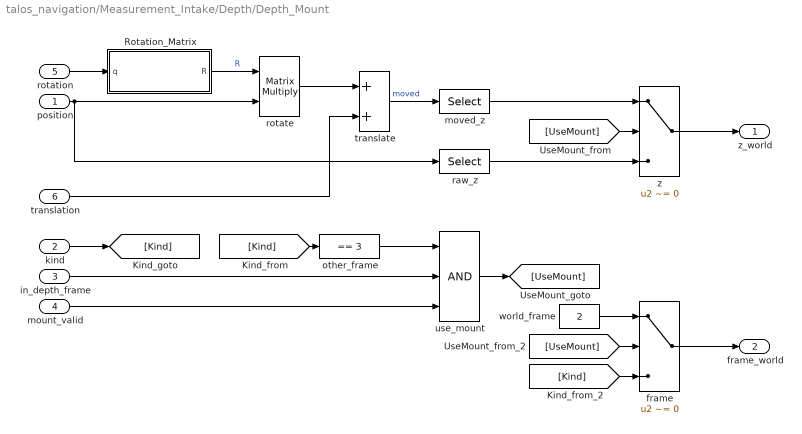
== system talos_navigation/Measurement_Intake/Depth/Depth_Mount ==
  position : Inport
  kind : Inport  Port=2
  in_depth_frame : Inport  Port=3
  mount_valid : Inport  Port=4
  rotation : Inport  Port=5
  translation : Inport  Port=6
  Rotation_Matrix : MATLAB Function  TreatAsAtomicUnit=on
  frame : Switch  Criteria=u2 ~= 0  SaturateOnIntegerOverflow=off  InputSameDT=off
  moved_z : Selector  InputPortWidth=3  IndexOptions=Index vector (dialog)  Indices=3  OutputSizes=1
  other_frame : simulink/Logic and Bit Operations/Compare To Constant  relop===  const=3  OutDataTypeStr=boolean
  raw_z : Selector  InputPortWidth=3  IndexOptions=Index vector (dialog)  Indices=3  OutputSizes=1
  rotate : Product  Multiplication=Matrix(*)
  translate : Sum
  use_mount : Logic  Inputs=3  AllPortsSameDT=off  OutDataTypeStr=boolean
  world_frame : Constant  Value=2
  z : Switch  Criteria=u2 ~= 0  SaturateOnIntegerOverflow=off  InputSameDT=off
  z_world : Outport
  frame_world : Outport  Port=2
  wires:
  rotation/1 -> Rotation_Matrix/1(q)
  Rotation_Matrix/1(R) -> rotate/1  "R"
  position/1 -> rotate/2, raw_z/1
  rotate/1 -> translate/1
  translation/1 -> translate/2
  translate/1 -> moved_z/1  "moved"
  moved_z/1 -> z/1
  raw_z/1 -> z/3
  kind/1 -> [Kind]
  [Kind] -> other_frame/1
  other_frame/1 -> use_mount/1
  in_depth_frame/1 -> use_mount/2
  mount_valid/1 -> use_mount/3
  use_mount/1 -> [UseMount]
  [UseMount] -> z/2
  [UseMount] -> frame/2
  [Kind] -> frame/3
  world_frame/1 -> frame/1
  z/1 -> z_world/1
  frame/1 -> frame_world/1

== system talos_navigation/Measurement_Intake/Depth/stamp ==
  stamp : Inport
  nanosec_int64 : DataTypeConversion  OutDataTypeStr=int64  SaturateOnIntegerOverflow=off  RndMeth=Floor
  parts : BusSelector  OutputSignals=sec,nanosec
  per_second : Gain  Gain=1000000000  ParamDataTypeStr=int64  OutDataTypeStr=int64
  sec_int64 : DataTypeConversion  OutDataTypeStr=int64  SaturateOnIntegerOverflow=off  RndMeth=Floor
  total : Sum  OutDataTypeStr=int64
  ns : Outport
  wires:
  stamp/1 -> parts/1
  parts/1 -> sec_int64/1  "<sec>"
  parts/2 -> nanosec_int64/1  "<nanosec>"
  sec_int64/1 -> per_second/1
  per_second/1 -> total/1
  nanosec_int64/1 -> total/2
  total/1 -> ns/1  "ns"

== system talos_navigation/Measurement_Intake/FOG/stamp ==
  stamp : Inport
  nanosec_int64 : DataTypeConversion  OutDataTypeStr=int64  SaturateOnIntegerOverflow=off  RndMeth=Floor
  parts : BusSelector  OutputSignals=sec,nanosec
  per_second : Gain  Gain=1000000000  ParamDataTypeStr=int64  OutDataTypeStr=int64
  sec_int64 : DataTypeConversion  OutDataTypeStr=int64  SaturateOnIntegerOverflow=off  RndMeth=Floor
  total : Sum  OutDataTypeStr=int64
  ns : Outport
  wires:
  stamp/1 -> parts/1
  parts/1 -> sec_int64/1  "<sec>"
  parts/2 -> nanosec_int64/1  "<nanosec>"
  sec_int64/1 -> per_second/1
  per_second/1 -> total/1
  nanosec_int64/1 -> total/2
  total/1 -> ns/1  "ns"

== system talos_navigation/Measurement_Intake/IMU/stamp ==
  stamp : Inport
  nanosec_int64 : DataTypeConversion  OutDataTypeStr=int64  SaturateOnIntegerOverflow=off  RndMeth=Floor
  parts : BusSelector  OutputSignals=sec,nanosec
  per_second : Gain  Gain=1000000000  ParamDataTypeStr=int64  OutDataTypeStr=int64
  sec_int64 : DataTypeConversion  OutDataTypeStr=int64  SaturateOnIntegerOverflow=off  RndMeth=Floor
  total : Sum  OutDataTypeStr=int64
  ns : Outport
  wires:
  stamp/1 -> parts/1
  parts/1 -> sec_int64/1  "<sec>"
  parts/2 -> nanosec_int64/1  "<nanosec>"
  sec_int64/1 -> per_second/1
  per_second/1 -> total/1
  nanosec_int64/1 -> total/2
  total/1 -> ns/1  "ns"

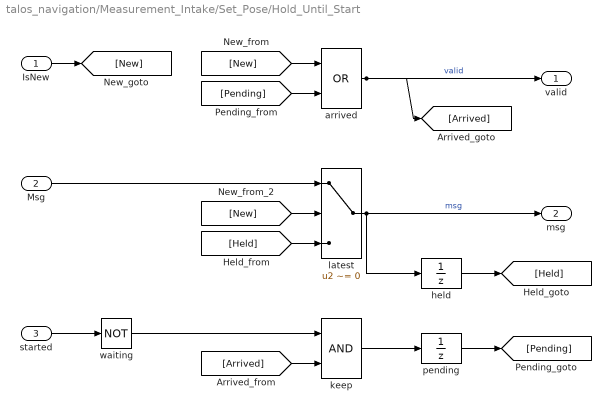
== system talos_navigation/Measurement_Intake/Set_Pose/Hold_Until_Start ==
  IsNew : Inport
  Msg : Inport  Port=2
  started : Inport  Port=3
  arrived : Logic  Operator=OR  AllPortsSameDT=off  OutDataTypeStr=boolean
  held : UnitDelay  SampleTime=-1  HasFrameUpgradeWarning=on
  keep : Logic  AllPortsSameDT=off  OutDataTypeStr=boolean
  latest : Switch  Criteria=u2 ~= 0  SaturateOnIntegerOverflow=off  InputSameDT=off
  pending : UnitDelay  InitialCondition=false  SampleTime=-1  HasFrameUpgradeWarning=on
  waiting : Logic  Operator=NOT  AllPortsSameDT=off  OutDataTypeStr=boolean
  valid : Outport
  msg : Outport  Port=2
  wires:
  IsNew/1 -> [New]
  [New] -> arrived/1
  [Pending] -> arrived/2
  arrived/1 -> valid/1, [Arrived]  "valid"
  [New] -> latest/2
  [Held] -> latest/3
  Msg/1 -> latest/1
  latest/1 -> msg/1, held/1  "msg"
  held/1 -> [Held]
  [Arrived] -> keep/2
  started/1 -> waiting/1
  waiting/1 -> keep/1
  keep/1 -> pending/1
  pending/1 -> [Pending]

== system talos_navigation/Measurement_Intake/Set_Pose/stamp ==
  stamp : Inport
  nanosec_int64 : DataTypeConversion  OutDataTypeStr=int64  SaturateOnIntegerOverflow=off  RndMeth=Floor
  parts : BusSelector  OutputSignals=sec,nanosec
  per_second : Gain  Gain=1000000000  ParamDataTypeStr=int64  OutDataTypeStr=int64
  sec_int64 : DataTypeConversion  OutDataTypeStr=int64  SaturateOnIntegerOverflow=off  RndMeth=Floor
  total : Sum  OutDataTypeStr=int64
  ns : Outport
  wires:
  stamp/1 -> parts/1
  parts/1 -> sec_int64/1  "<sec>"
  parts/2 -> nanosec_int64/1  "<nanosec>"
  sec_int64/1 -> per_second/1
  per_second/1 -> total/1
  nanosec_int64/1 -> total/2
  total/1 -> ns/1  "ns"

== system talos_navigation/Parameters/estimator/imu_acceleration_bias ==
  element_0 : ros2lib/Get Parameter  ParameterName=navigation__estimator__imu_acceleration_bias_0  ParameterType=double  ParameterMaxArrayLength=16  ParameterInitialValue=0  SampleTime=1/10.0  ModelName=ros2lib  BlockId=ParamGet_ros2lib_196
  element_1 : ros2lib/Get Parameter  ParameterName=navigation__estimator__imu_acceleration_bias_1  ParameterType=double  ParameterMaxArrayLength=16  ParameterInitialValue=0  SampleTime=1/10.0  ModelName=ros2lib  BlockId=ParamGet_ros2lib_196
  element_2 : ros2lib/Get Parameter  ParameterName=navigation__estimator__imu_acceleration_bias_2  ParameterType=double  ParameterMaxArrayLength=16  ParameterInitialValue=-0.044545  SampleTime=1/10.0  ModelName=ros2lib  BlockId=ParamGet_ros2lib_196
  elements : Concatenate  NumInputs=3
  value : Outport
  wires:
  element_0/1 -> elements/1
  element_1/1 -> elements/2
  element_2/1 -> elements/3
  elements/1 -> value/1
